simulink model "model_Silnika"  (Simulink 6.3)
settings: Solver=ode45  StartTime=0.0  StopTime=1000  RelTol=1e-3
settings Model: LastModifiedBy=GLOWEK

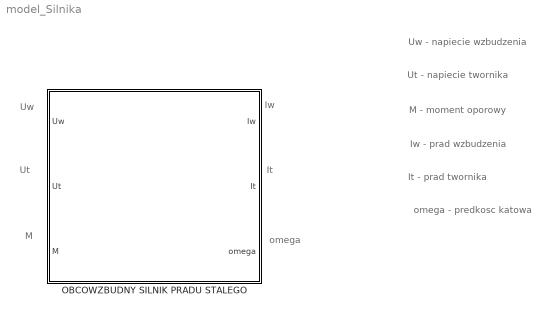
== system model_Silnika ==
  note: Uw
  note: Ut
  note: M
  note: Iw
  note: It
  note: omega
  note: Uw - napiecie wzbudzenia
  note: Ut - napiecie twornika
  note: M - moment oporowy
  note: Iw - prad wzbudzenia
  note: It - prad twornika
  note: omega - predkosc katowa
  OBCOWZBUDNY SILNIK PRADU STALEGO : Subsystem
      mask init:
      | [data, map]=imread('silnik.gif');
      | pic=ind2rgb(data,map);
      mask Display: image(pic)

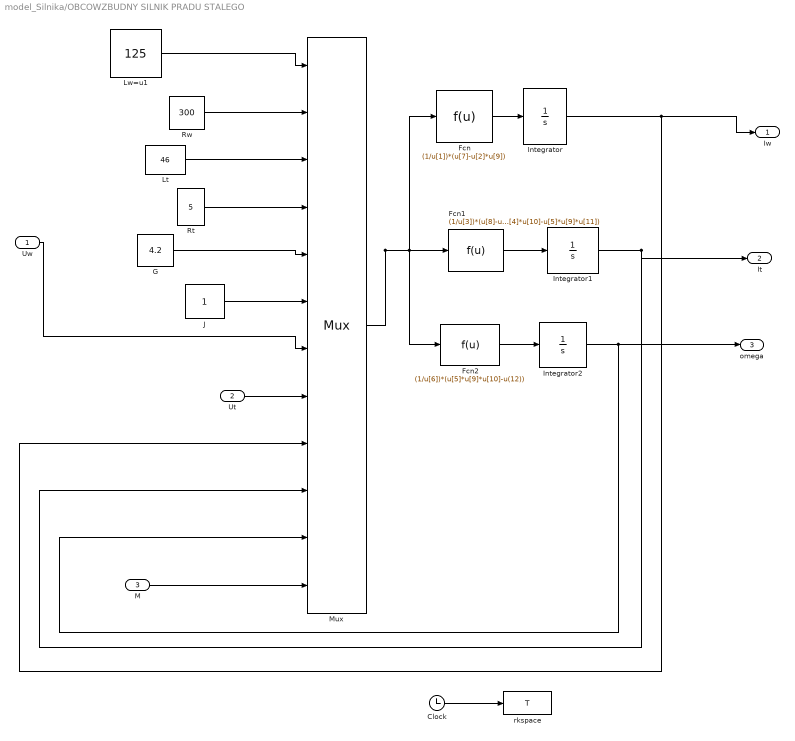
== system model_Silnika/OBCOWZBUDNY SILNIK PRADU STALEGO ==
  Uw : Inport
  Ut : Inport  Port=2
  M : Inport  Port=3
  Clock : Clock
      settings: Decimation=10
  Fcn : Fcn  Expr=(1/u[1])*(u[7]-u[2]*u[9])
  Fcn1 : Fcn  Expr=(1/u[3])*(u[8]-u[4]*u[10]-u[5]*u[9]*u[11])
  Fcn2 : Fcn  Expr=(1/u[6])*(u[5]*u[9]*u[10]-u(12))
  G : Constant  Value=4.2
  Integrator : Integrator
  Integrator1 : Integrator
  Integrator2 : Integrator
  J : Constant
  Lt : Constant  Value=46
  Lw=u1 : Constant  Value=125
  Mux : Mux  Inputs=12
  Rt : Constant  Value=5
  Rw : Constant  Value=300
  rkspace : ToWorkspace  VariableName=T  SampleTime=-1  SaveFormat=Array
  Iw : Outport
  It : Outport  Port=2
  omega : Outport  Port=3
  wires:
  Lw=u1/1 -> Mux/1
  Rw/1 -> Mux/2
  Lt/1 -> Mux/3
  J/1 -> Mux/6
  Fcn/1 -> Integrator/1
  Fcn1/1 -> Integrator1/1
  Rt/1 -> Mux/4
  Integrator/1 -> Mux/9, Iw/1
  Integrator1/1 -> Mux/10, It/1
  Fcn2/1 -> Integrator2/1
  Integrator2/1 -> Mux/11, omega/1
  Mux/1 -> Fcn/1, Fcn1/1, Fcn2/1
  G/1 -> Mux/5
  Clock/1 -> rkspace/1
  Uw/1 -> Mux/7
  M/1 -> Mux/12
  Ut/1 -> Mux/8
